simulink model "IEEE_BUS_68_Baseline"  (R2025a)
settings: Solver=ode23tb  StartTime=0.0  StopTime=150  FixedStep=Ts  MaxStep=0.0001  RelTol=1e-3
PreLoadFcn:
  | PSSMODEL=1;
  | LPSS=0;
  | WAPSS=0;
  | WAPSS2=0;
  | Ts=50e-5;
InitFcn:
  | PSSMODEL=1;
  | LPSS=0;
  | WAPSS=0;
  | WAPSS2=0;
  | Ts=50e-5;
  | 
  | % Required data to 68 Bus benchmark
  | % clear
  | % clc
  | % Definition for the columns
  | % system base =100 MVA
  | 
  | %% Line data Format (line)
  | % All values are given on the same system base MVA
  | % 1: From bus
  | % 2: To bus
  | % 3: Resistance (pu)
  | % 4: Reactance  (pu)
  | % 5: Charge     (pu)
  | % 6: Transformer Tap Amplitute
  | % 7: base MVA
  | % 8: Nomonal Voltage (KV)
  | 
  | %1   2    3        4       5       6        7      8
  | line=[...
  | 1	54	0	     0.0181	  0	      1.025     100    13.8
  | 2	58	0	     0.025	  0	      1.070     100    13.8
  | 3	62	0	     0.02	  0	      1.070     100    13.8
  | 4	19	0.0007	 0.0142	  0	      1.070     100    13.8
  | 5	20	0.0009	 0.018	  0	      1.009     100    13.8
  | 6	22	0	     0.0143	  0	      1.025     100    13.8
  | 7	23	0.0005	 0.0272	  0	      0         100    13.8
  | 8	25	0.0006	 0.0232	  0	      1.025     100    13.8
  | 9	29	0.0008	 0.0156   0	      1.025     100    13.8
  | 10	31	0	     0.026	  0	      1.04      100    13.8
  | 11	32	0	     0.013	  0	      1.04      100    13.8
  | 12	36	0	     0.0075	  0	      1.04      100    13.8
  | 13	17	0	     0.0033	  0	      1.04      100    13.8
  | 14	41	0	     0.0015	  0	      1         100    13.8
  | 15	42	0	     0.0015	  0	      1         100    13.8
  | 16	18	0	     0.003	  0	      1         100    13.8
  | 17	36	0.0005	 0.0045	  0.32	  0         100    138
  | 17	43	0.0005	 0.0276	  0	      0         100    138
  | 18	42	0.004	 0.06	  2.25    0         100    138
  | 18	49	0.0076	 0.1141	  1.16    0	        100    138
  | 18	50	0.0012	 0.0288	  2.06	  0         100    138
  | 20	19	0.0007	 0.0138	  0       1.06	    100    138
  | 19	68	0.0016	 0.0195	  0.304	  0         100    138
  | 21	22	0.0008	 0.014	  0.2565  0	        100    138
  | 21	68	0.0008	 0.0135	  0.2548  0	        100    138
  | 22	23	0.0006	 0.0096	  0.1846  0	        100    138
  | 23	24	0.0022	 0.035	  0.361	  0         100    138
  | 24	68	0.0003	 0.0059	  0.068	  0         100    138
  | 25	26	0.0032	 0.0323	  0.531	  0         100    138
  | 25	54	0.007	 0.0086	  0.146	  0         100    138
  | 26	27	0.0014	 0.0147	  0.2396  0	        100    138
  | 26	28	0.0043	 0.0474	  0.7802  0	        100    138
  | 26	29	0.0057	 0.0625	  1.029	  0         100    138
  | 27	37	0.0013	 0.0173	  0.3216  0	        100    138
  | 27	53	0.032	 0.32	  0.41	  0         100    138
  | ... (+206 lines)
undefined symbols (not defined in the file or in its folder): D1, Delta
libraries: spsRMSLib x73, spsThreePhaseVIMeasurementLib x69, spsLoadFlowBusLib x69, spsThreePhasePISectionLineLib x64, spsThreePhaseParallelRLCLoadLib x35, spsGenericPowerSystemStabilizerLib x32, spsThreePhaseSeriesRLCLoadLib x21, spsThreePhaseTransformerTwoWindingsLib x21, spsSynchronousMachinepuStandardLib x19, spsExcitationSystemLib x16, spsMultiBandPowerSystemStabilizerLib x16, spsSteamTurbineandGovernorLib x16
(part 5 of 7)

== system IEEE_BUS_68_Baseline/area-3/G1 ==
  "M1: Turbine & Regulators " : Subsystem
  Pref1 : Constant  Value=0.25
  Vref1 : Constant  Value=1.045
  gen1 : spsSynchronousMachinepuStandardLib/Synchronous Machine pu Standard  PresetModel=No  MechanicalLoad=Mechanical power Pm  ShowDetailedParameters=on  RotorType=Round  Units=per unit standard parameters  MeasurementBus=off  NominalParameters="[1000*1e6  13.8e3  60 ]"  Reactances1="[mac_con(1,6:8)  mac_con(1,11:13)  mac_con(1,4)]"  Reactances2=[ 1.305, 0.296, 0.252, 0.474, 0.243, 0.18 ]  dAxisTimeConstants=Open-circuit  qAxisTimeConstants=Open-circuit  TimeConstants1=[]  TimeConstants2="[mac_con(1,9:10)  mac_con(1,14:15)]"  TimeConstants3=[]  TimeConstants4=[]  TimeConstants5=[ 1.01, 0.053, 0.1 ]  TimeConstants6=[]  TimeConstants7=[]  TimeConstants8=[]  StatorResistance=mac_con(1,5)  Mechanical="[ mac_con(1,16)  0  4]"  PolePairs=4  InitialConditions=[0 -92.3264 0.281269 0.281269 0.281269 -34.9508 -154.951 85.0492 1.06004]  SetSaturation=off  Saturation=[0.6404,0.7127,0.8441,0.9214,0.9956,1.082,1.19,1.316,1.457;0.7,0.7698,0.8872,0.9466,0.9969,1.046,1.1,1.151,1.201]  LoadFlowParameters=[1 830000000 0 0 0]  TsPowergui=0  TsBlock=-1  IterativeModel=Trapezoidal non iterative  IterativeDiscreteModel=Trapezoidal non iterative  BusType=PV  Pref=250000000  Qref=0  Qmin=-Inf  Qmax=Inf  PLF=0  QLF=0
  A : PMIOPort  Side=Left
  B : PMIOPort  Port=2  Side=Left
  C : PMIOPort  Port=3  Side=Left
  wires:
  Vref1/1 -> "M1: Turbine & Regulators "/3(Vref1)
  [PSSmodel] -> "M1: Turbine & Regulators "/4(PSS1)
  gen1/1 -> "M1: Turbine & Regulators "/1(m1)
  "M1: Turbine & Regulators "/2(Vf1) -> gen1/2
  "M1: Turbine & Regulators "/1(Pm1) -> gen1/1
  Pref1/1 -> "M1: Turbine & Regulators "/2(Pref1)
  connections:
  C/RConn1 -- gen1/RConn3
  B/RConn1 -- gen1/RConn2
  A/RConn1 -- gen1/RConn1

== system IEEE_BUS_68_Baseline/area-3/G8 ==
  "M8: Turbine & Regulators " : Subsystem
  Pref8 : Constant  Value=0.54
  Vref8 : Constant  Value=1.03
  gen8 : spsSynchronousMachinepuStandardLib/Synchronous Machine pu Standard  PresetModel=No  MechanicalLoad=Mechanical power Pm  ShowDetailedParameters=on  RotorType=Round  Units=per unit standard parameters  MeasurementBus=off  NominalParameters="[1000*1e6  13.8e3   60 ]"  Reactances1="[mac_con(8,6:8)  mac_con(8,11:13)  mac_con(8,4)]"  Reactances2=[ 1.305, 0.296, 0.252, 0.474, 0.243, 0.18 ]  dAxisTimeConstants=Open-circuit  qAxisTimeConstants=Open-circuit  TimeConstants1=[]  TimeConstants2="[mac_con(8,9:10)  mac_con(8,14:15)]"  TimeConstants3=[]  TimeConstants4=[]  TimeConstants5=[ 1.01, 0.053, 0.1 ]  TimeConstants6=[]  TimeConstants7=[]  TimeConstants8=[]  StatorResistance=mac_con(8,5)  Mechanical="[ mac_con(8,16)  0  4]"  PolePairs=4  InitialConditions=[0 -79.3312 0.524289 0.524289 0.524289 2.10404 -117.896 122.104 1.04236]  SetSaturation=off  Saturation=[0.6404,0.7127,0.8441,0.9214,0.9956,1.082,1.19,1.316,1.457;0.7,0.7698,0.8872,0.9466,0.9969,1.046,1.1,1.151,1.201]  LoadFlowParameters=[1 830000000 0 0 0]  TsPowergui=0  TsBlock=-1  IterativeModel=Trapezoidal non iterative  IterativeDiscreteModel=Trapezoidal non iterative  BusType=PV  Pref=540000000  Qref=0  Qmin=-Inf  Qmax=Inf  PLF=0  QLF=0
  A : PMIOPort  Side=Left
  B : PMIOPort  Port=2  Side=Left
  C : PMIOPort  Port=3  Side=Left
  wires:
  Pref8/1 -> "M8: Turbine & Regulators "/2(Pref8)
  "M8: Turbine & Regulators "/1(Pm8) -> gen8/1
  "M8: Turbine & Regulators "/2(Vf8) -> gen8/2
  gen8/1 -> "M8: Turbine & Regulators "/1(m8)
  [PSSmodel] -> "M8: Turbine & Regulators "/4(PSS8)
  Vref8/1 -> "M8: Turbine & Regulators "/3(Vref8)
  connections:
  A/RConn1 -- gen8/RConn1
  B/RConn1 -- gen8/RConn2
  C/RConn1 -- gen8/RConn3

== system IEEE_BUS_68_Baseline/area-3/G9 ==
  "M9: Turbine & Regulators " : Subsystem
  Pref9 : Constant  Value=0.8
  Vref9 : Constant  Value=1.025
  gen9 : spsSynchronousMachinepuStandardLib/Synchronous Machine pu Standard  PresetModel=No  MechanicalLoad=Mechanical power Pm  ShowDetailedParameters=on  RotorType=Round  Units=per unit standard parameters  MeasurementBus=off  NominalParameters="[1000*1e6  13.8e3   60 ]"  Reactances1="[mac_con(9,6:8)  mac_con(9,11:13)  mac_con(9,4)]"  Reactances2=[ 1.305, 0.296, 0.252, 0.474, 0.243, 0.18 ]  dAxisTimeConstants=Open-circuit  qAxisTimeConstants=Open-circuit  TimeConstants1=[]  TimeConstants2="[mac_con(9,9:10)  mac_con(9,14:15)]"  TimeConstants3=[]  TimeConstants4=[]  TimeConstants5=[ 1.01, 0.053, 0.1 ]  TimeConstants6=[]  TimeConstants7=[]  TimeConstants8=[]  StatorResistance=mac_con(9,5)  Mechanical="[ mac_con(9,16)  0  4]"  PolePairs=4  InitialConditions=[0 -77.9749 0.781129 0.781129 0.781129 0.886411 -119.114 120.886 1.04467]  SetSaturation=off  Saturation=[0.6404,0.7127,0.8441,0.9214,0.9956,1.082,1.19,1.316,1.457;0.7,0.7698,0.8872,0.9466,0.9969,1.046,1.1,1.151,1.201]  LoadFlowParameters=[1 830000000 0 0 0]  TsPowergui=0  TsBlock=-1  IterativeModel=Trapezoidal non iterative  IterativeDiscreteModel=Trapezoidal non iterative  BusType=PV  Pref=800000000  Qref=0  Qmin=-Inf  Qmax=Inf  PLF=0  QLF=0
  A : PMIOPort  Side=Left
  B : PMIOPort  Port=2  Side=Left
  C : PMIOPort  Port=3  Side=Left
  wires:
  Vref9/1 -> "M9: Turbine & Regulators "/3(Vref9)
  [PSSmodel] -> "M9: Turbine & Regulators "/4(PSS9)
  gen9/1 -> "M9: Turbine & Regulators "/1(m9)
  "M9: Turbine & Regulators "/2(Vf9) -> gen9/2
  "M9: Turbine & Regulators "/1(Pm9) -> gen9/1
  Pref9/1 -> "M9: Turbine & Regulators "/2(Pref9)
  connections:
  C/RConn1 -- gen9/RConn3
  B/RConn1 -- gen9/RConn2
  A/RConn1 -- gen9/RConn1

== system IEEE_BUS_68_Baseline/area-4/G10 ==
  "M10: Turbine & Regulators " : Subsystem
  Pref10 : Constant  Value=0.5
  Vref10 : Constant  Value=1.01
  gen10 : spsSynchronousMachinepuStandardLib/Synchronous Machine pu Standard  PresetModel=No  MechanicalLoad=Mechanical power Pm  ShowDetailedParameters=on  RotorType=Round  Units=per unit standard parameters  MeasurementBus=off  NominalParameters="[1000*1e6  13.8e3   60 ]"  Reactances1="[mac_con(10,6:8)  mac_con(10,11:13)  mac_con(10,4)]"  Reactances2=[ 1.305, 0.296, 0.252, 0.474, 0.243, 0.18 ]  dAxisTimeConstants=Open-circuit  qAxisTimeConstants=Open-circuit  TimeConstants1=[]  TimeConstants2="[mac_con(10,9:10)  mac_con(10,14:15)]"  TimeConstants3=[]  TimeConstants4=[]  TimeConstants5=[ 1.01, 0.053, 0.1 ]  TimeConstants6=[]  TimeConstants7=[]  TimeConstants8=[]  StatorResistance=mac_con(10,5)  Mechanical="[ mac_con(10,16)  0  4]"  PolePairs=4  InitialConditions=[0 -89.8437 0.495254 0.495254 0.495254 -4.71293 -124.713 115.287 1.01551]  SetSaturation=off  Saturation=[0.6404,0.7127,0.8441,0.9214,0.9956,1.082,1.19,1.316,1.457;0.7,0.7698,0.8872,0.9466,0.9969,1.046,1.1,1.151,1.201]  LoadFlowParameters=[1 830000000 0 0 0]  TsPowergui=0  TsBlock=-1  IterativeModel=Trapezoidal non iterative  IterativeDiscreteModel=Trapezoidal non iterative  BusType=PV  Pref=500000000  Qref=0  Qmin=-Inf  Qmax=Inf  PLF=0  QLF=0
  A : PMIOPort  Side=Left
  B : PMIOPort  Port=2  Side=Left
  C : PMIOPort  Port=3  Side=Left
  wires:
  Vref10/1 -> "M10: Turbine & Regulators "/3(Vref10)
  [PSSmodel] -> "M10: Turbine & Regulators "/4(PSS10)
  gen10/1 -> "M10: Turbine & Regulators "/1(m10)
  "M10: Turbine & Regulators "/2(Vf10) -> gen10/2
  "M10: Turbine & Regulators "/1(Pm10) -> gen10/1
  Pref10/1 -> "M10: Turbine & Regulators "/2(Pref10)
  connections:
  C/RConn1 -- gen10/RConn3
  B/RConn1 -- gen10/RConn2
  A/RConn1 -- gen10/RConn1

== system IEEE_BUS_68_Baseline/area-4/G11 ==
  "M11: Turbine & Regulators " : Subsystem
  Pref11 : Constant  Value=0.5
  Vref11 : Constant
  gen11 : spsSynchronousMachinepuStandardLib/Synchronous Machine pu Standard  PresetModel=No  MechanicalLoad=Mechanical power Pm  ShowDetailedParameters=on  RotorType=Round  Units=per unit standard parameters  MeasurementBus=off  NominalParameters="[2000*1e6  13.8e3   60 ]"  Reactances1="[mac_con(11,6:8)  mac_con(11,11:13)  mac_con(11,4)]"  Reactances2=[ 1.305, 0.296, 0.252, 0.474, 0.243, 0.18 ]  dAxisTimeConstants=Open-circuit  qAxisTimeConstants=Open-circuit  TimeConstants1=[]  TimeConstants2="[mac_con(11,9:10)  mac_con(11,14:15)]"  TimeConstants3=[]  TimeConstants4=[]  TimeConstants5=[ 1.01, 0.053, 0.1 ]  TimeConstants6=[]  TimeConstants7=[]  TimeConstants8=[]  StatorResistance=mac_con(11,5)  Mechanical="[ mac_con(11,16)  0  4]"  PolePairs=4  InitialConditions=[0 -88.1407 0.500589 0.500589 0.500589 -4.42976 -124.43 115.57 1.00514]  SetSaturation=off  Saturation=[0.6404,0.7127,0.8441,0.9214,0.9956,1.082,1.19,1.316,1.457;0.7,0.7698,0.8872,0.9466,0.9969,1.046,1.1,1.151,1.201]  LoadFlowParameters=[1 830000000 0 0 0]  TsPowergui=0  TsBlock=-1  IterativeModel=Trapezoidal non iterative  IterativeDiscreteModel=Trapezoidal non iterative  BusType=PV  Pref=1000000000  Qref=0  Qmin=-Inf  Qmax=Inf  PLF=0  QLF=0
  A : PMIOPort  Side=Left
  B : PMIOPort  Port=2  Side=Left
  C : PMIOPort  Port=3  Side=Left
  wires:
  Pref11/1 -> "M11: Turbine & Regulators "/2(Pref11)
  "M11: Turbine & Regulators "/1(Pm11) -> gen11/1
  "M11: Turbine & Regulators "/2(Vf11) -> gen11/2
  gen11/1 -> "M11: Turbine & Regulators "/1(m11)
  [PSSmodel] -> "M11: Turbine & Regulators "/4(PSS11)
  Vref11/1 -> "M11: Turbine & Regulators "/3(Vref11)
  connections:
  A/RConn1 -- gen11/RConn1
  B/RConn1 -- gen11/RConn2
  C/RConn1 -- gen11/RConn3

== system IEEE_BUS_68_Baseline/area-4/G12 ==
  "M12: Turbine & Regulators " : Subsystem
  Pref12 : Constant  Value=0.45
  Vref12 : Constant  Value=1.0156
  gen12 : spsSynchronousMachinepuStandardLib/Synchronous Machine pu Standard  PresetModel=No  MechanicalLoad=Mechanical power Pm  ShowDetailedParameters=on  RotorType=Round  Units=per unit standard parameters  MeasurementBus=off  NominalParameters="[3000*1e6  13.8e3   60 ]"  Reactances1="[mac_con(12,6:8)  mac_con(12,11:13)  mac_con(12,4)]"  Reactances2=[ 1.305, 0.296, 0.252, 0.474, 0.243, 0.18 ]  dAxisTimeConstants=Open-circuit  qAxisTimeConstants=Open-circuit  TimeConstants1=[]  TimeConstants2="[mac_con(12,9:10)  mac_con(12,14:15)]"  TimeConstants3=[]  TimeConstants4=[]  TimeConstants5=[ 1.01, 0.053, 0.1 ]  TimeConstants6=[]  TimeConstants7=[]  TimeConstants8=[]  StatorResistance=mac_con(12,5)  Mechanical="[ mac_con(12,16)  0  4]"  PolePairs=4  InitialConditions=[0 -102.326 0.444178 0.444178 0.444178 -10.6913 -130.691 109.309 1.01344]  SetSaturation=off  Saturation=[0.6404,0.7127,0.8441,0.9214,0.9956,1.082,1.19,1.316,1.457;0.7,0.7698,0.8872,0.9466,0.9969,1.046,1.1,1.151,1.201]  LoadFlowParameters=[1 830000000 0 0 0]  TsPowergui=0  TsBlock=-1  IterativeModel=Trapezoidal non iterative  IterativeDiscreteModel=Trapezoidal non iterative  BusType=PV  Pref=1350000000  Qref=0  Qmin=-Inf  Qmax=Inf  PLF=0  QLF=0
  A : PMIOPort  Side=Left
  B : PMIOPort  Port=2  Side=Left
  C : PMIOPort  Port=3  Side=Left
  wires:
  Vref12/1 -> "M12: Turbine & Regulators "/3(Vref12)
  [PSSmodel] -> "M12: Turbine & Regulators "/4(PSS12)
  gen12/1 -> "M12: Turbine & Regulators "/1(m12)
  "M12: Turbine & Regulators "/2(Vf12) -> gen12/2
  "M12: Turbine & Regulators "/1(Pm12) -> gen12/1
  Pref12/1 -> "M12: Turbine & Regulators "/2(Pref12)
  connections:
  C/RConn1 -- gen12/RConn3
  B/RConn1 -- gen12/RConn2
  A/RConn1 -- gen12/RConn1

== system IEEE_BUS_68_Baseline/area-4/G13 ==
  "M11: Turbine & Regulators " : Subsystem
  Pref13 : Constant  Value=0.5985
  Vref13 : Constant  Value=1.011
  gen13 : spsSynchronousMachinepuStandardLib/Synchronous Machine pu Standard  PresetModel=No  MechanicalLoad=Mechanical power Pm  ShowDetailedParameters=on  RotorType=Round  Units=per unit standard parameters  MeasurementBus=off  NominalParameters="[6000*1e6  13.8e3   60 ]"  Reactances1="[mac_con(13,6:8)  mac_con(13,11:13)  mac_con(13,4)]"  Reactances2=[ 1.305, 0.296, 0.252, 0.474, 0.243, 0.18 ]  dAxisTimeConstants=Open-circuit  qAxisTimeConstants=Open-circuit  TimeConstants1=[]  TimeConstants2="[mac_con(13,9:10)  mac_con(13,14:15)]"  TimeConstants3=[]  TimeConstants4=[]  TimeConstants5=[ 1.01, 0.053, 0.1 ]  TimeConstants6=[]  TimeConstants7=[]  TimeConstants8=[]  StatorResistance=mac_con(13,5)  Mechanical="[ mac_con(13,16)  0  4]"  PolePairs=4  InitialConditions=[0 -109.135 0.613282 0.613282 0.613282 -35.2324 -155.232 84.7676 1.01589]  SetSaturation=off  Saturation=[0.6404,0.7127,0.8441,0.9214,0.9956,1.082,1.19,1.316,1.457;0.7,0.7698,0.8872,0.9466,0.9969,1.046,1.1,1.151,1.201]  LoadFlowParameters=[1 830000000 0 0 0]  TsPowergui=0  TsBlock=-1  IterativeModel=Trapezoidal non iterative  IterativeDiscreteModel=Trapezoidal non iterative  BusType=PV  Pref=3591000000  Qref=0  Qmin=-Inf  Qmax=Inf  PLF=0  QLF=0
  A : PMIOPort  Side=Left
  B : PMIOPort  Port=2  Side=Left
  C : PMIOPort  Port=3  Side=Left
  wires:
  Pref13/1 -> "M11: Turbine & Regulators "/2(Pref13)
  "M11: Turbine & Regulators "/1(Pm13) -> gen13/1
  "M11: Turbine & Regulators "/2(Vf13) -> gen13/2
  gen13/1 -> "M11: Turbine & Regulators "/1(m13)
  [PSSmodel] -> "M11: Turbine & Regulators "/4(PSS13)
  Vref13/1 -> "M11: Turbine & Regulators "/3(Vref13)
  connections:
  A/RConn1 -- gen13/RConn1
  B/RConn1 -- gen13/RConn2
  C/RConn1 -- gen13/RConn3

== system IEEE_BUS_68_Baseline/area-5/G14 ==
  "M14: Turbine & Regulators " : Subsystem
  Pref14 : Constant  Value=0.595
  Vref14 : Constant
  gen14 : spsSynchronousMachinepuStandardLib/Synchronous Machine pu Standard  PresetModel=No  MechanicalLoad=Mechanical power Pm  ShowDetailedParameters=on  RotorType=Round  Units=per unit standard parameters  MeasurementBus=off  NominalParameters="[3000*1e6  13.8e3   60 ]"  Reactances1="[mac_con(14,6:8)  mac_con(14,11:13)  mac_con(14,4)]"  Reactances2=[ 1.305, 0.296, 0.252, 0.474, 0.243, 0.18 ]  dAxisTimeConstants=Open-circuit  qAxisTimeConstants=Open-circuit  TimeConstants1=[]  TimeConstants2="[mac_con(14,9:10)  mac_con(14,14:15)]"  TimeConstants3=[]  TimeConstants4=[]  TimeConstants5=[ 1.01, 0.053, 0.1 ]  TimeConstants6=[]  TimeConstants7=[]  TimeConstants8=[]  StatorResistance=mac_con(14,5)  Mechanical="[ mac_con(14,16)  0  4]"  PolePairs=4  InitialConditions=[0 -72.2334 0.595447 0.595447 0.595447 14.9563 -105.044 134.956 1.00047]  SetSaturation=off  Saturation=[0.6404,0.7127,0.8441,0.9214,0.9956,1.082,1.19,1.316,1.457;0.7,0.7698,0.8872,0.9466,0.9969,1.046,1.1,1.151,1.201]  LoadFlowParameters=[1 830000000 0 0 0]  TsPowergui=0  TsBlock=-1  IterativeModel=Trapezoidal non iterative  IterativeDiscreteModel=Trapezoidal non iterative  BusType=PV  Pref=1785000000  Qref=0  Qmin=-Inf  Qmax=Inf  PLF=0  QLF=0
  A : PMIOPort  Side=Left
  B : PMIOPort  Port=2  Side=Left
  C : PMIOPort  Port=3  Side=Left
  wires:
  Vref14/1 -> "M14: Turbine & Regulators "/3(Vref14)
  [PSSmodel] -> "M14: Turbine & Regulators "/4(PSS14)
  gen14/1 -> "M14: Turbine & Regulators "/1(m14)
  "M14: Turbine & Regulators "/2(Vf14) -> gen14/2
  "M14: Turbine & Regulators "/1(Pm14) -> gen14/1
  Pref14/1 -> "M14: Turbine & Regulators "/2(Pref14)
  connections:
  C/RConn1 -- gen14/RConn3
  B/RConn1 -- gen14/RConn2
  A/RConn1 -- gen14/RConn1

== system IEEE_BUS_68_Baseline/area-5/G15 ==
  "M15: Turbine & Regulators " : Subsystem
  Pref15 : Constant  Value=0.33333
  Vref15 : Constant
  gen15 : spsSynchronousMachinepuStandardLib/Synchronous Machine pu Standard  PresetModel=No  MechanicalLoad=Mechanical power Pm  ShowDetailedParameters=on  RotorType=Round  Units=per unit standard parameters  MeasurementBus=off  NominalParameters="[3000*1e6  13.8e3   60 ]"  Reactances1="[mac_con(15,6:8)  mac_con(15,11:13)  mac_con(15,4)]"  Reactances2=[ 1.305, 0.296, 0.252, 0.474, 0.243, 0.18 ]  dAxisTimeConstants=Open-circuit  qAxisTimeConstants=Open-circuit  TimeConstants1=[]  TimeConstants2="[mac_con(15,9:10)  mac_con(15,14:15)]"  TimeConstants3=[]  TimeConstants4=[]  TimeConstants5=[ 1.01, 0.053, 0.1 ]  TimeConstants6=[]  TimeConstants7=[]  TimeConstants8=[]  StatorResistance=mac_con(15,5)  Mechanical="[ mac_con(15,16)  0  4]"  PolePairs=4  InitialConditions=[0 -83.6244 0.334246 0.334246 0.334246 1.81112 -118.189 121.811 1.00046]  SetSaturation=off  Saturation=[0.6404,0.7127,0.8441,0.9214,0.9956,1.082,1.19,1.316,1.457;0.7,0.7698,0.8872,0.9466,0.9969,1.046,1.1,1.151,1.201]  LoadFlowParameters=[1 830000000 0 0 0]  TsPowergui=0  TsBlock=-1  IterativeModel=Trapezoidal non iterative  IterativeDiscreteModel=Trapezoidal non iterative  BusType=PV  Pref=1000000000  Qref=0  Qmin=-Inf  Qmax=Inf  PLF=0  QLF=0
  A : PMIOPort  Side=Left
  B : PMIOPort  Port=2  Side=Left
  C : PMIOPort  Port=3  Side=Left
  wires:
  Pref15/1 -> "M15: Turbine & Regulators "/2(Pref15)
  "M15: Turbine & Regulators "/1(Pm15) -> gen15/1
  "M15: Turbine & Regulators "/2(Vf15) -> gen15/2
  gen15/1 -> "M15: Turbine & Regulators "/1(m15)
  [PSSmodel] -> "M15: Turbine & Regulators "/4(PSS15)
  Vref15/1 -> "M15: Turbine & Regulators "/3(Vref15)
  connections:
  A/RConn1 -- gen15/RConn1
  B/RConn1 -- gen15/RConn2
  C/RConn1 -- gen15/RConn3

== system IEEE_BUS_68_Baseline/area-5/G16 ==
  "M16: Turbine & Regulators " : Subsystem
  Pref16 : Constant  Value=0.58333
  Vref16 : Constant
  gen16 : spsSynchronousMachinepuStandardLib/Synchronous Machine pu Standard  PresetModel=No  MechanicalLoad=Mechanical power Pm  ShowDetailedParameters=on  RotorType=Round  Units=per unit standard parameters  MeasurementBus=off  NominalParameters="[6000*1e6  13.8e3   60 ]"  Reactances1="[mac_con(13,6:8)  mac_con(13,11:13)  mac_con(13,4)]"  Reactances2=[ 1.305, 0.296, 0.252, 0.474, 0.243, 0.18 ]  dAxisTimeConstants=Open-circuit  qAxisTimeConstants=Open-circuit  TimeConstants1=[]  TimeConstants2="[mac_con(13,9:10)  mac_con(13,14:15)]"  TimeConstants3=[]  TimeConstants4=[]  TimeConstants5=[ 1.01, 0.053, 0.1 ]  TimeConstants6=[]  TimeConstants7=[]  TimeConstants8=[]  StatorResistance=mac_con(13,5)  Mechanical="[ mac_con(13,16)  0  4]"  PolePairs=4  InitialConditions=[0 -83.032 0.584666 0.584666 0.584666 2.14369 -117.856 122.144 1.00132]  SetSaturation=off  Saturation=[0.6404,0.7127,0.8441,0.9214,0.9956,1.082,1.19,1.316,1.457;0.7,0.7698,0.8872,0.9466,0.9969,1.046,1.1,1.151,1.201]  LoadFlowParameters=[1 830000000 0 0 0]  TsPowergui=0  TsBlock=-1  IterativeModel=Trapezoidal non iterative  IterativeDiscreteModel=Trapezoidal non iterative  BusType=PV  Pref=3500000000  Qref=0  Qmin=-Inf  Qmax=Inf  PLF=0  QLF=0
  A : PMIOPort  Side=Left
  B : PMIOPort  Port=2  Side=Left
  C : PMIOPort  Port=3  Side=Left
  wires:
  Vref16/1 -> "M16: Turbine & Regulators "/3(Vref16)
  [PSSmodel] -> "M16: Turbine & Regulators "/4(PSS16)
  gen16/1 -> "M16: Turbine & Regulators "/1(m16)
  "M16: Turbine & Regulators "/2(Vf16) -> gen16/2
  "M16: Turbine & Regulators "/1(Pm16) -> gen16/1
  Pref16/1 -> "M16: Turbine & Regulators "/2(Pref16)
  connections:
  C/RConn1 -- gen16/RConn3
  B/RConn1 -- gen16/RConn2
  A/RConn1 -- gen16/RConn1

== system IEEE_BUS_68_Baseline/area-1/gen4/M4: Turbine & Regulators  ==
  note: M4
  m4 : Inport
  Pref4 : Inport  Port=2
  Vref4 : Inport  Port=3
  PSS4 : Inport  Port=4
  Bus Selector : BusSelector  OutputSignals="Mechanical.Rotor speed  wm  (pu),Mechanical.Rotor angle deviation  d_theta (rad),Mechanical.Electrical power  Pe (pu),Mechanical.Rotor speed deviation  dw (pu),Mechanical.Rotor mechanical angle  theta (deg),dq0 components.Stator voltage  vd (pu),dq0 components.Stator voltage  vq (pu),Output reactive power  Qeo (pu)"
  Delta Pa PSS 4 : spsGenericPowerSystemStabilizerLib/Generic Power System Stabilizer  Tsensor=15e-3  K=2.5*1.25  Twashout=1  Tleadlag1=[60e-3 1]  Tleadlag2=[0 0]  VSlimits=[-0.15 0.15]  Vinit=0  Plot_On=off  MagdB_On=on  FreqRange=logspace(-2,2,500)
      settings: LibrarySourceBlock=|
      | sps_lib/Electrical Machines/Synchronous Machine Control/Generic
      | Power System Stabilizer
  Delta w PSS (Kundur) 4 : spsGenericPowerSystemStabilizerLib/Generic Power System Stabilizer  Tsensor=15e-3  K=30  Twashout=10  Tleadlag1=[50e-3 20e-3]  Tleadlag2=[3 5.4]  VSlimits=[-0.15 0.15]  Vinit=0  Plot_On=off  MagdB_On=on  FreqRange=logspace(-2,2,500)
      settings: LibrarySourceBlock=|
      | sps_lib/Electrical Machines/Synchronous Machine Control/Generic
      | Power System Stabilizer
  EXCITATION4 : spsExcitationSystemLib/Excitation System  tr=AVR_Data(4,1)  reg=[ AVR_Data(4,2:3) ]  exc=[ 1, 0 ]  tgr=[ AVR_Data(4,4:5)]  damp=[ 0, 0 ]  sat=[ 0, 0 ]  lim="[ AVR_Data(4,7:8)  0 ]"  v0=[0.997 1.0061]
      settings: LibrarySourceBlock=sps_lib/Electrical Machines/Synchronous Machine Control/Excitation System
  MB-PSS4 : spsMultiBandPowerSystemStabilizerLib/Multi-Band Power System Stabilizer  OperationMode=Simplified settings  Kg=MB(1)  GL=[MB(2) MB(3)]  GI=[MB(4) MB(5)]  GH=[MB(6) MB(7)]  GLd=[66 66 9.4]  TcLF=[1.667 2 0 0 0 0 2 2.4 0 0 0 0 1 1]  GId=[66 66 47.6]  TcIF=[1 1 0.25 0.3 0 0 1 1 0.3 0.36 0 0 0 0]  GHd=[66 66 233]  TcHF="[0.01 0.012 0 0 0 0  0.012 0.0144 0 0 0 0 1 1]"  LIM=[.075 .15 .15 .15]  Plot_On=off  MagdB_On=off  FreqRange=logspace(-2,2,500)
      settings: LibrarySourceBlock=|
      | sps_lib/Electrical Machines/Synchronous Machine Control/Multi-Band
      | Power System Stabilizer
  Multiport Switch1 : MultiPortSwitch  Inputs=4  SaturateOnIntegerOverflow=off
  PSS model3 : Constant  Value=0
  PSS model4 : Constant
  Real-Imag to Complex1 : RealImagToComplex
  STG4 : spsSteamTurbineandGovernorLib/Steam Turbine and Governor  gentype=Tandem-compound (single mass)  reg1="[ 1  0.05    0 ]"  reg2="[ 0.001  0.15 ]"  reg3="[ -0.1  0.1  0  4.496 ]"  N=Ns  turb1="[ 0  10   3.3   0.5   ]"  turb2="[   0   0.36    0.36   0.28   ]"  HA="[ 0.046  1.430  1.465   0.192 ]"  KA="[ 90.44  53.88  64.59   62.94  ]"  DA="[ 0.0115  0.3575  0.3663   0.0137  ]"  ini1=0.632  ini2=[0.779316,-31.4247]
      settings: LibrarySourceBlock=|
      | sps_lib/Electrical Machines/Synchronous Machine Control/Steam Turbine
      | and Governor
  Sum2 : Sum  InputSameDT=on  SaturateOnIntegerOverflow=on  OutDataTypeStr=Inherit: Same as first input
  Sum3 : Sum  Inputs=-+  InputSameDT=on  SaturateOnIntegerOverflow=on  OutDataTypeStr=Inherit: Same as first input
  Terminator3 : Terminator
  Terminator4 : Terminator
  Terminator5 : Terminator
  wref4 : Constant
  Pm4 : Outport  InitialOutput=0
  Vf4 : Outport  Port=2  InitialOutput=0
  tag scope: EFD4=global, Pa4=global, Pe4=global, Q4=global, Vt4=global, d_theta4=global, pss4=global, theta4=global, w4=global
  wires:
  Bus Selector/7 -> EXCITATION4/3, Real-Imag to Complex1/2  "<Stator voltage  vq (pu)>"
  wref4/1 -> STG4/1
  Pref4/1 -> STG4/2
  m4/1 -> Bus Selector/1
  Vref4/1 -> EXCITATION4/1
  EXCITATION4/1 -> Vf4/1, [EFD4]
  Real-Imag to Complex1/1 -> [Vt4]
  Bus Selector/5 -> [theta4]  "<Rotor mechanical angle  theta (deg)>"
  Bus Selector/6 -> EXCITATION4/2, Real-Imag to Complex1/1  "<Stator voltage  vd (pu)>"
  STG4/3 -> Terminator3/1
  STG4/4 -> Sum3/2, Pm4/1
  STG4/2 -> Terminator4/1
  STG4/1 -> Terminator5/1
  Bus Selector/1 -> [w4], STG4/3  "<Rotor speed  wm  (pu)>"
  Bus Selector/2 -> STG4/4, [d_theta4]  "<Rotor angle deviation  d_theta (rad)>"
  Bus Selector/3 -> Sum3/1, [Pe4]  "<Electrical power  Pe (pu)>"
  Bus Selector/4 -> Delta w PSS (Kundur) 4/1, MB-PSS4/1  "<Rotor speed deviation  dw (pu)>"
  Bus Selector/8 -> [Q4]  "<Output reactive power  Qeo (pu)>"
  Sum3/1 -> [Pa4], Delta Pa PSS 4/1  "Pm-Pe"
  Sum2/1 -> Multiport Switch1/1
  PSS model4/1 -> Sum2/2
  Delta Pa PSS 4/1 -> Multiport Switch1/5
  Delta w PSS (Kundur) 4/1 -> Multiport Switch1/4
  MB-PSS4/1 -> Multiport Switch1/3
  PSS model3/1 -> Multiport Switch1/2
  Multiport Switch1/1 -> [pss4], EXCITATION4/4
  PSS4/1 -> Sum2/1

== system IEEE_BUS_68_Baseline/area-1/gen5/M4: Turbine & Regulators  ==
  note: M5
  m5 : Inport
  Pref5 : Inport  Port=2
  Vref5 : Inport  Port=3
  PSS5 : Inport  Port=4
  Bus Selector : BusSelector  OutputSignals="Mechanical.Rotor speed  wm  (pu),Mechanical.Rotor angle deviation  d_theta (rad),Mechanical.Electrical power  Pe (pu),Mechanical.Rotor speed deviation  dw (pu),Mechanical.Rotor mechanical angle  theta (deg),dq0 components.Stator voltage  vd (pu),dq0 components.Stator voltage  vq (pu),Output reactive power  Qeo (pu)"
  Delta Pa PSS 5 : spsGenericPowerSystemStabilizerLib/Generic Power System Stabilizer  Tsensor=15e-3  K=2.5*1.25  Twashout=1  Tleadlag1=[60e-3 1]  Tleadlag2=[0 0]  VSlimits=[-0.15 0.15]  Vinit=0  Plot_On=off  MagdB_On=on  FreqRange=logspace(-2,2,500)
      settings: LibrarySourceBlock=|
      | sps_lib/Electrical Machines/Synchronous Machine Control/Generic
      | Power System Stabilizer
  Delta w PSS (Kundur) 5 : spsGenericPowerSystemStabilizerLib/Generic Power System Stabilizer  Tsensor=15e-3  K=30  Twashout=10  Tleadlag1=[50e-3 20e-3]  Tleadlag2=[3 5.4]  VSlimits=[-0.15 0.15]  Vinit=0  Plot_On=off  MagdB_On=on  FreqRange=logspace(-2,2,500)
      settings: LibrarySourceBlock=|
      | sps_lib/Electrical Machines/Synchronous Machine Control/Generic
      | Power System Stabilizer
  EXCITATION5 : spsExcitationSystemLib/Excitation System  tr=AVR_Data(4,1)  reg=[ AVR_Data(4,2:3) ]  exc=[ 1, 0 ]  tgr=[ AVR_Data(4,4:5)]  damp=[ 0, 0 ]  sat=[ 0, 0 ]  lim="[ AVR_Data(4,7:8)  0 ]"  v0=[1.011 1.0594]
      settings: LibrarySourceBlock=sps_lib/Electrical Machines/Synchronous Machine Control/Excitation System
  MB-PSS5 : spsMultiBandPowerSystemStabilizerLib/Multi-Band Power System Stabilizer  OperationMode=Simplified settings  Kg=MB(1)  GL=[MB(2) MB(3)]  GI=[MB(4) MB(5)]  GH=[MB(6) MB(7)]  GLd=[66 66 9.4]  TcLF=[1.667 2 0 0 0 0 2 2.4 0 0 0 0 1 1]  GId=[66 66 47.6]  TcIF=[1 1 0.25 0.3 0 0 1 1 0.3 0.36 0 0 0 0]  GHd=[66 66 233]  TcHF="[0.01 0.012 0 0 0 0  0.012 0.0144 0 0 0 0 1 1]"  LIM=[.075 .15 .15 .15]  Plot_On=off  MagdB_On=off  FreqRange=logspace(-2,2,500)
      settings: LibrarySourceBlock=|
      | sps_lib/Electrical Machines/Synchronous Machine Control/Multi-Band
      | Power System Stabilizer
  Multiport Switch1 : MultiPortSwitch  Inputs=4  SaturateOnIntegerOverflow=off
  PSS model3 : Constant  Value=0
  PSS model4 : Constant
  Real-Imag to Complex1 : RealImagToComplex
  STG5 : spsSteamTurbineandGovernorLib/Steam Turbine and Governor  gentype=Tandem-compound (single mass)  reg1="[ 1  0.05    0 ]"  reg2="[ 0.001  0.15 ]"  reg3="[ -0.1  0.1  0  4.496 ]"  N=Ns  turb1="[ 0  10   3.3   0.5   ]"  turb2="[   0   0.36    0.36   0.28   ]"  HA="[ 0.046  1.430  1.465   0.192 ]"  KA="[ 90.44  53.88  64.59   62.94  ]"  DA="[ 0.0115  0.3575  0.3663   0.0137  ]"  ini1=0.505  ini2=[0.779316,-31.4247]
      settings: LibrarySourceBlock=|
      | sps_lib/Electrical Machines/Synchronous Machine Control/Steam Turbine
      | and Governor
  Sum2 : Sum  InputSameDT=on  SaturateOnIntegerOverflow=on  OutDataTypeStr=Inherit: Same as first input
  Sum3 : Sum  Inputs=-+  InputSameDT=on  SaturateOnIntegerOverflow=on  OutDataTypeStr=Inherit: Same as first input
  Terminator3 : Terminator
  Terminator4 : Terminator
  Terminator5 : Terminator
  wref5 : Constant
  Pm4 : Outport  InitialOutput=0
  Vf5 : Outport  Port=2  InitialOutput=0
  tag scope: EFD5=global, Pa5=global, Pe5=global, Q5=global, Vt5=global, d_theta5=global, pss5=global, theta5=global, w5=global
  wires:
  PSS5/1 -> Sum2/1
  Multiport Switch1/1 -> EXCITATION5/4, [pss5]
  PSS model3/1 -> Multiport Switch1/2
  MB-PSS5/1 -> Multiport Switch1/3
  Delta w PSS (Kundur) 5/1 -> Multiport Switch1/4
  Delta Pa PSS 5/1 -> Multiport Switch1/5
  PSS model4/1 -> Sum2/2
  Sum2/1 -> Multiport Switch1/1
  Sum3/1 -> Delta Pa PSS 5/1, [Pa5]  "Pm-Pe"
  Bus Selector/8 -> [Q5]  "<Output reactive power  Qeo (pu)>"
  Bus Selector/4 -> MB-PSS5/1, Delta w PSS (Kundur) 5/1  "<Rotor speed deviation  dw (pu)>"
  Bus Selector/3 -> [Pe5], Sum3/1  "<Electrical power  Pe (pu)>"
  Bus Selector/2 -> [d_theta5], STG5/4  "<Rotor angle deviation  d_theta (rad)>"
  Bus Selector/1 -> STG5/3, [w5]  "<Rotor speed  wm  (pu)>"
  STG5/1 -> Terminator5/1
  STG5/2 -> Terminator4/1
  STG5/4 -> Pm4/1, Sum3/2
  STG5/3 -> Terminator3/1
  Bus Selector/6 -> Real-Imag to Complex1/1, EXCITATION5/2  "<Stator voltage  vd (pu)>"
  Bus Selector/5 -> [theta5]  "<Rotor mechanical angle  theta (deg)>"
  Real-Imag to Complex1/1 -> [Vt5]
  EXCITATION5/1 -> [EFD5], Vf5/1
  Vref5/1 -> EXCITATION5/1
  m5/1 -> Bus Selector/1
  Pref5/1 -> STG5/2
  wref5/1 -> STG5/1
  Bus Selector/7 -> Real-Imag to Complex1/2, EXCITATION5/3  "<Stator voltage  vq (pu)>"

== system IEEE_BUS_68_Baseline/area-1/gen6/M4: Turbine & Regulators  ==
  note: M6
  m6 : Inport
  Pref6 : Inport  Port=2
  Vref6 : Inport  Port=3
  PSS6 : Inport  Port=4
  Bus Selector : BusSelector  OutputSignals="Mechanical.Rotor speed  wm  (pu),Mechanical.Rotor angle deviation  d_theta (rad),Mechanical.Electrical power  Pe (pu),Mechanical.Rotor speed deviation  dw (pu),Mechanical.Rotor mechanical angle  theta (deg),dq0 components.Stator voltage  vd (pu),dq0 components.Stator voltage  vq (pu),Output reactive power  Qeo (pu)"
  Delta Pa PSS 6 : spsGenericPowerSystemStabilizerLib/Generic Power System Stabilizer  Tsensor=15e-3  K=2.5*1.25  Twashout=1  Tleadlag1=[60e-3 1]  Tleadlag2=[0 0]  VSlimits=[-0.15 0.15]  Vinit=0  Plot_On=off  MagdB_On=on  FreqRange=logspace(-2,2,500)
      settings: LibrarySourceBlock=|
      | sps_lib/Electrical Machines/Synchronous Machine Control/Generic
      | Power System Stabilizer
  Delta w PSS (Kundur) 6 : spsGenericPowerSystemStabilizerLib/Generic Power System Stabilizer  Tsensor=15e-3  K=30  Twashout=10  Tleadlag1=[50e-3 20e-3]  Tleadlag2=[3 5.4]  VSlimits=[-0.15 0.15]  Vinit=0  Plot_On=off  MagdB_On=on  FreqRange=logspace(-2,2,500)
      settings: LibrarySourceBlock=|
      | sps_lib/Electrical Machines/Synchronous Machine Control/Generic
      | Power System Stabilizer
  EXCITATION6 : spsExcitationSystemLib/Excitation System  tr=AVR_Data(4,1)  reg=[ AVR_Data(4,2:3) ]  exc=[ 1, 0 ]  tgr=[ AVR_Data(4,4:5)]  damp=[ 0, 0 ]  sat=[ 0, 0 ]  lim="[ AVR_Data(4,7:8)  0 ]"  v0=[1.05 1.1031]
      settings: LibrarySourceBlock=sps_lib/Electrical Machines/Synchronous Machine Control/Excitation System
  MB-PSS6 : spsMultiBandPowerSystemStabilizerLib/Multi-Band Power System Stabilizer  OperationMode=Simplified settings  Kg=MB(1)  GL=[MB(2) MB(3)]  GI=[MB(4) MB(5)]  GH=[MB(6) MB(7)]  GLd=[66 66 9.4]  TcLF=[1.667 2 0 0 0 0 2 2.4 0 0 0 0 1 1]  GId=[66 66 47.6]  TcIF=[1 1 0.25 0.3 0 0 1 1 0.3 0.36 0 0 0 0]  GHd=[66 66 233]  TcHF="[0.01 0.012 0 0 0 0  0.012 0.0144 0 0 0 0 1 1]"  LIM=[.075 .15 .15 .15]  Plot_On=off  MagdB_On=off  FreqRange=logspace(-2,2,500)
      settings: LibrarySourceBlock=|
      | sps_lib/Electrical Machines/Synchronous Machine Control/Multi-Band
      | Power System Stabilizer
  Multiport Switch1 : MultiPortSwitch  Inputs=4  SaturateOnIntegerOverflow=off
  PSS model3 : Constant  Value=0
  PSS model4 : Constant
  Real-Imag to Complex1 : RealImagToComplex
  STG6 : spsSteamTurbineandGovernorLib/Steam Turbine and Governor  gentype=Tandem-compound (single mass)  reg1="[ 1  0.05    0 ]"  reg2="[ 0.001  0.15 ]"  reg3="[ -0.1  0.1  0  4.496 ]"  N=Ns  turb1="[ 0  10   3.3   0.5   ]"  turb2="[   0   0.36    0.36   0.28   ]"  HA="[ 0.046  1.430  1.465   0.192 ]"  KA="[ 90.44  53.88  64.59   62.94  ]"  DA="[ 0.0115  0.3575  0.3663   0.0137  ]"  ini1=0.7  ini2=[0.779316,-31.4247]
      settings: LibrarySourceBlock=|
      | sps_lib/Electrical Machines/Synchronous Machine Control/Steam Turbine
      | and Governor
  Sum2 : Sum  InputSameDT=on  SaturateOnIntegerOverflow=on  OutDataTypeStr=Inherit: Same as first input
  Sum3 : Sum  Inputs=-+  InputSameDT=on  SaturateOnIntegerOverflow=on  OutDataTypeStr=Inherit: Same as first input
  Terminator3 : Terminator
  Terminator4 : Terminator
  Terminator5 : Terminator
  wref6 : Constant
  Pm6 : Outport  InitialOutput=0
  Vf6 : Outport  Port=2  InitialOutput=0
  tag scope: EFD6=global, Pa6=global, Pe6=global, Q6=global, Vt6=global, d_theta6=global, pss6=global, theta6=global, w6=global
  wires:
  PSS6/1 -> Sum2/1
  Multiport Switch1/1 -> EXCITATION6/4, [pss6]
  PSS model3/1 -> Multiport Switch1/2
  MB-PSS6/1 -> Multiport Switch1/3
  Delta w PSS (Kundur) 6/1 -> Multiport Switch1/4
  Delta Pa PSS 6/1 -> Multiport Switch1/5
  PSS model4/1 -> Sum2/2
  Sum2/1 -> Multiport Switch1/1
  Sum3/1 -> Delta Pa PSS 6/1, [Pa6]  "Pm-Pe"
  Bus Selector/8 -> [Q6]  "<Output reactive power  Qeo (pu)>"
  Bus Selector/4 -> MB-PSS6/1, Delta w PSS (Kundur) 6/1  "<Rotor speed deviation  dw (pu)>"
  Bus Selector/3 -> [Pe6], Sum3/1  "<Electrical power  Pe (pu)>"
  Bus Selector/2 -> [d_theta6], STG6/4  "<Rotor angle deviation  d_theta (rad)>"
  Bus Selector/1 -> STG6/3, [w6]  "<Rotor speed  wm  (pu)>"
  STG6/1 -> Terminator5/1
  STG6/2 -> Terminator4/1
  STG6/4 -> Pm6/1, Sum3/2
  STG6/3 -> Terminator3/1
  Bus Selector/6 -> Real-Imag to Complex1/1, EXCITATION6/2  "<Stator voltage  vd (pu)>"
  Bus Selector/5 -> [theta6]  "<Rotor mechanical angle  theta (deg)>"
  Real-Imag to Complex1/1 -> [Vt6]
  EXCITATION6/1 -> [EFD6], Vf6/1
  Vref6/1 -> EXCITATION6/1
  m6/1 -> Bus Selector/1
  Pref6/1 -> STG6/2
  wref6/1 -> STG6/1
  Bus Selector/7 -> Real-Imag to Complex1/2, EXCITATION6/3  "<Stator voltage  vq (pu)>"

== system IEEE_BUS_68_Baseline/area-1/gen7/M7: Turbine & Regulators  ==
  note: M7
  m7 : Inport
  Pref7 : Inport  Port=2
  Vref7 : Inport  Port=3
  PSS7 : Inport  Port=4
  Bus Selector : BusSelector  OutputSignals="Mechanical.Rotor speed  wm  (pu),Mechanical.Rotor angle deviation  d_theta (rad),Mechanical.Electrical power  Pe (pu),Mechanical.Rotor speed deviation  dw (pu),Mechanical.Rotor mechanical angle  theta (deg),dq0 components.Stator voltage  vd (pu),dq0 components.Stator voltage  vq (pu),Output reactive power  Qeo (pu)"
  Delta Pa PSS 7 : spsGenericPowerSystemStabilizerLib/Generic Power System Stabilizer  Tsensor=15e-3  K=2.5*1.25  Twashout=1  Tleadlag1=[60e-3 1]  Tleadlag2=[0 0]  VSlimits=[-0.15 0.15]  Vinit=0  Plot_On=off  MagdB_On=on  FreqRange=logspace(-2,2,500)
      settings: LibrarySourceBlock=|
      | sps_lib/Electrical Machines/Synchronous Machine Control/Generic
      | Power System Stabilizer
  Delta w PSS (Kundur) 7 : spsGenericPowerSystemStabilizerLib/Generic Power System Stabilizer  Tsensor=15e-3  K=30  Twashout=10  Tleadlag1=[50e-3 20e-3]  Tleadlag2=[3 5.4]  VSlimits=[-0.15 0.15]  Vinit=0  Plot_On=off  MagdB_On=on  FreqRange=logspace(-2,2,500)
      settings: LibrarySourceBlock=|
      | sps_lib/Electrical Machines/Synchronous Machine Control/Generic
      | Power System Stabilizer
  EXCITATION7 : spsExcitationSystemLib/Excitation System  tr=AVR_Data(4,1)  reg=[ AVR_Data(4,2:3) ]  exc=[ 1, 0 ]  tgr=[ AVR_Data(4,4:5)]  damp=[ 0, 0 ]  sat=[ 0, 0 ]  lim="[ AVR_Data(4,7:8)  0 ]"  v0=[1.063 1.1186]
      settings: LibrarySourceBlock=sps_lib/Electrical Machines/Synchronous Machine Control/Excitation System
  MB-PSS7 : spsMultiBandPowerSystemStabilizerLib/Multi-Band Power System Stabilizer  OperationMode=Simplified settings  Kg=MB(1)  GL=[MB(2) MB(3)]  GI=[MB(4) MB(5)]  GH=[MB(6) MB(7)]  GLd=[66 66 9.4]  TcLF=[1.667 2 0 0 0 0 2 2.4 0 0 0 0 1 1]  GId=[66 66 47.6]  TcIF=[1 1 0.25 0.3 0 0 1 1 0.3 0.36 0 0 0 0]  GHd=[66 66 233]  TcHF="[0.01 0.012 0 0 0 0  0.012 0.0144 0 0 0 0 1 1]"  LIM=[.075 .15 .15 .15]  Plot_On=off  MagdB_On=off  FreqRange=logspace(-2,2,500)
      settings: LibrarySourceBlock=|
      | sps_lib/Electrical Machines/Synchronous Machine Control/Multi-Band
      | Power System Stabilizer
  Multiport Switch1 : MultiPortSwitch  Inputs=4  SaturateOnIntegerOverflow=off
  PSS model3 : Constant  Value=0
  PSS model4 : Constant
  Real-Imag to Complex1 : RealImagToComplex
  STG7 : spsSteamTurbineandGovernorLib/Steam Turbine and Governor  gentype=Tandem-compound (single mass)  reg1="[ 1  0.05    0 ]"  reg2="[ 0.001  0.15 ]"  reg3="[ -0.1  0.1  0  4.496 ]"  N=Ns  turb1="[ 0  10   3.3   0.5   ]"  turb2="[   0   0.36    0.36   0.28   ]"  HA="[ 0.046  1.430  1.465   0.192 ]"  KA="[ 90.44  53.88  64.59   62.94  ]"  DA="[ 0.0115  0.3575  0.3663   0.0137  ]"  ini1=0.56  ini2=[0.779316,-31.4247]
      settings: LibrarySourceBlock=|
      | sps_lib/Electrical Machines/Synchronous Machine Control/Steam Turbine
      | and Governor
  Sum2 : Sum  InputSameDT=on  SaturateOnIntegerOverflow=on  OutDataTypeStr=Inherit: Same as first input
  Sum3 : Sum  Inputs=-+  InputSameDT=on  SaturateOnIntegerOverflow=on  OutDataTypeStr=Inherit: Same as first input
  Terminator3 : Terminator
  Terminator4 : Terminator
  Terminator5 : Terminator
  wref7 : Constant
  Pm7 : Outport  InitialOutput=0
  Vf7 : Outport  Port=2  InitialOutput=0
  tag scope: EFD7=global, Pa7=global, Pe7=global, Q7=global, Vt7=global, d_theta7=global, pss7=global, theta7=global, w7=global
  wires:
  PSS7/1 -> Sum2/1
  Multiport Switch1/1 -> EXCITATION7/4, [pss7]
  PSS model3/1 -> Multiport Switch1/2
  MB-PSS7/1 -> Multiport Switch1/3
  Delta w PSS (Kundur) 7/1 -> Multiport Switch1/4
  Delta Pa PSS 7/1 -> Multiport Switch1/5
  PSS model4/1 -> Sum2/2
  Sum2/1 -> Multiport Switch1/1
  Sum3/1 -> Delta Pa PSS 7/1, [Pa7]  "Pm-Pe"
  Bus Selector/8 -> [Q7]  "<Output reactive power  Qeo (pu)>"
  Bus Selector/4 -> MB-PSS7/1, Delta w PSS (Kundur) 7/1  "<Rotor speed deviation  dw (pu)>"
  Bus Selector/3 -> [Pe7], Sum3/1  "<Electrical power  Pe (pu)>"
  Bus Selector/2 -> [d_theta7], STG7/4  "<Rotor angle deviation  d_theta (rad)>"
  Bus Selector/1 -> STG7/3, [w7]  "<Rotor speed  wm  (pu)>"
  STG7/1 -> Terminator5/1
  STG7/2 -> Terminator4/1
  STG7/4 -> Pm7/1, Sum3/2
  STG7/3 -> Terminator3/1
  Bus Selector/6 -> Real-Imag to Complex1/1, EXCITATION7/2  "<Stator voltage  vd (pu)>"
  Bus Selector/5 -> [theta7]  "<Rotor mechanical angle  theta (deg)>"
  Real-Imag to Complex1/1 -> [Vt7]
  EXCITATION7/1 -> [EFD7], Vf7/1
  Vref7/1 -> EXCITATION7/1
  m7/1 -> Bus Selector/1
  Pref7/1 -> STG7/2
  wref7/1 -> STG7/1
  Bus Selector/7 -> Real-Imag to Complex1/2, EXCITATION7/3  "<Stator voltage  vq (pu)>"

== system IEEE_BUS_68_Baseline/area-2/G2/M2: Turbine & Regulators  ==
  note: M2
  m2 : Inport
  Pref2 : Inport  Port=2
  Vref2 : Inport  Port=3
  PSS2 : Inport  Port=4
  Bus Selector : BusSelector  OutputSignals="Mechanical.Rotor speed  wm  (pu),Mechanical.Rotor angle deviation  d_theta (rad),Mechanical.Electrical power  Pe (pu),Mechanical.Rotor speed deviation  dw (pu),Mechanical.Rotor mechanical angle  theta (deg),dq0 components.Stator voltage  vd (pu),dq0 components.Stator voltage  vq (pu),Output reactive power  Qeo (pu)"
  "Delta Pa PSS 2 " : spsGenericPowerSystemStabilizerLib/Generic Power System Stabilizer  Tsensor=15e-3  K=2.5*1.25  Twashout=1  Tleadlag1=[60e-3 1]  Tleadlag2=[0 0]  VSlimits=[-0.15 0.15]  Vinit=0  Plot_On=off  MagdB_On=on  FreqRange=logspace(-2,2,500)
      settings: LibrarySourceBlock=|
      | sps_lib/Electrical Machines/Synchronous Machine Control/Generic
      | Power System Stabilizer
  Delta w PSS (Kundur) 2 : spsGenericPowerSystemStabilizerLib/Generic Power System Stabilizer  Tsensor=15e-3  K=30  Twashout=10  Tleadlag1=[50e-3 20e-3]  Tleadlag2=[3 5.4]  VSlimits=[-0.15 0.15]  Vinit=0  Plot_On=off  MagdB_On=on  FreqRange=logspace(-2,2,500)
      settings: LibrarySourceBlock=|
      | sps_lib/Electrical Machines/Synchronous Machine Control/Generic
      | Power System Stabilizer
  EXCITATION2 : spsExcitationSystemLib/Excitation System  tr=AVR_Data(2,1)  reg=[ AVR_Data(2,2:3) ]  exc=[ 1, 0 ]  tgr=[ AVR_Data(2,4:5)]  damp=[ 0, 0 ]  sat=[ 0, 0 ]  lim="[ AVR_Data(2,7:8)  0 ]"  v0=[0.98 1.0211]
      settings: LibrarySourceBlock=sps_lib/Electrical Machines/Synchronous Machine Control/Excitation System
  MB-PSS2 : spsMultiBandPowerSystemStabilizerLib/Multi-Band Power System Stabilizer  OperationMode=Simplified settings  Kg=MB(1)  GL=[MB(2) MB(3)]  GI=[MB(4) MB(5)]  GH=[MB(6) MB(7)]  GLd=[66 66 9.4]  TcLF=[1.667 2 0 0 0 0 2 2.4 0 0 0 0 1 1]  GId=[66 66 47.6]  TcIF=[1 1 0.25 0.3 0 0 1 1 0.3 0.36 0 0 0 0]  GHd=[66 66 233]  TcHF="[0.01 0.012 0 0 0 0  0.012 0.0144 0 0 0 0 1 1]"  LIM=[.075 .15 .15 .15]  Plot_On=off  MagdB_On=off  FreqRange=logspace(-2,2,500)
      settings: LibrarySourceBlock=|
      | sps_lib/Electrical Machines/Synchronous Machine Control/Multi-Band
      | Power System Stabilizer
  Multiport Switch1 : MultiPortSwitch  Inputs=4  SaturateOnIntegerOverflow=off
  PSS model3 : Constant  Value=0
  PSS model4 : Constant
  Real-Imag to Complex1 : RealImagToComplex
  STG2 : spsSteamTurbineandGovernorLib/Steam Turbine and Governor  gentype=Tandem-compound (single mass)  reg1="[ 1  0.05    0 ]"  reg2="[ 0.001  0.15 ]"  reg3="[ -0.1  0.1  0  4.496 ]"  N=Ns  turb1="[ 0  10   3.3   0.5   ]"  turb2="[   0   0.36    0.36   0.28   ]"  HA="[ 0.046  1.430  1.465   0.192 ]"  KA="[ 90.44  53.88  64.59   62.94  ]"  DA="[ 0.0115  0.3575  0.3663   0.0137  ]"  ini1=0.545  ini2=[0.779316,-31.4247]
      settings: LibrarySourceBlock=|
      | sps_lib/Electrical Machines/Synchronous Machine Control/Steam Turbine
      | and Governor
  Sum2 : Sum  InputSameDT=on  SaturateOnIntegerOverflow=on  OutDataTypeStr=Inherit: Same as first input
  Sum3 : Sum  Inputs=-+  InputSameDT=on  SaturateOnIntegerOverflow=on  OutDataTypeStr=Inherit: Same as first input
  Terminator3 : Terminator
  Terminator4 : Terminator
  Terminator5 : Terminator
  wref2 : Constant
  Pm2 : Outport  InitialOutput=0
  Vf2 : Outport  Port=2  InitialOutput=0
  tag scope: EFD2=global, Pa2=global, Pe2=global, Q2=global, Vt2=global, d_theta2=global, pss2=global, theta2=global, w2=global
  wires:
  Bus Selector/7 -> EXCITATION2/3, Real-Imag to Complex1/2  "<Stator voltage  vq (pu)>"
  wref2/1 -> STG2/1
  Pref2/1 -> STG2/2
  m2/1 -> Bus Selector/1
  Vref2/1 -> EXCITATION2/1
  EXCITATION2/1 -> Vf2/1, [EFD2]
  Real-Imag to Complex1/1 -> [Vt2]
  Bus Selector/5 -> [theta2]  "<Rotor mechanical angle  theta (deg)>"
  Bus Selector/6 -> EXCITATION2/2, Real-Imag to Complex1/1  "<Stator voltage  vd (pu)>"
  STG2/3 -> Terminator3/1
  STG2/4 -> Sum3/2, Pm2/1
  STG2/2 -> Terminator4/1
  STG2/1 -> Terminator5/1
  Bus Selector/1 -> [w2], STG2/3  "<Rotor speed  wm  (pu)>"
  Bus Selector/2 -> STG2/4, [d_theta2]  "<Rotor angle deviation  d_theta (rad)>"
  Bus Selector/3 -> Sum3/1, [Pe2]  "<Electrical power  Pe (pu)>"
  Bus Selector/4 -> Delta w PSS (Kundur) 2/1, MB-PSS2/1  "<Rotor speed deviation  dw (pu)>"
  Bus Selector/8 -> [Q2]  "<Output reactive power  Qeo (pu)>"
  Sum3/1 -> [Pa2], "Delta Pa PSS 2 "/1  "Pm-Pe"
  Sum2/1 -> Multiport Switch1/1
  PSS model4/1 -> Sum2/2
  "Delta Pa PSS 2 "/1 -> Multiport Switch1/5
  Delta w PSS (Kundur) 2/1 -> Multiport Switch1/4
  MB-PSS2/1 -> Multiport Switch1/3
  PSS model3/1 -> Multiport Switch1/2
  Multiport Switch1/1 -> [pss2], EXCITATION2/4
  PSS2/1 -> Sum2/1
